simulink model "pmsm_align"  (R2023b)
settings: Solver=FixedStepDiscrete  StartTime=0.0  StopTime=0.05  FixedStep=1e-5  RelTol=1e-3
values from neighbouring files (symbols this model uses):
  V = out.flog.signals.values    [add_ident2.m]    (also in add_w.m; add_w2.m; baseline_model.m; check_kt.m = out.mlog.signals.values)
libraries: spsControlledVoltageSourceLib x3, spsPermanentMagnetSynchronousMachineLib x1, spspowerguiLib x1
settings Model: Creator=28447  LastModifiedBy=28447

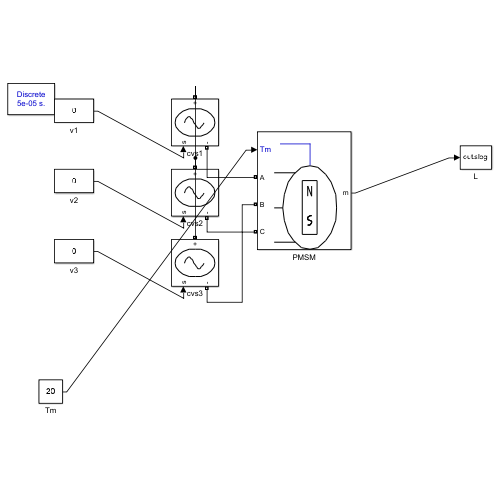
[thumbnail: Simulink's stored preview of the top-level diagram]
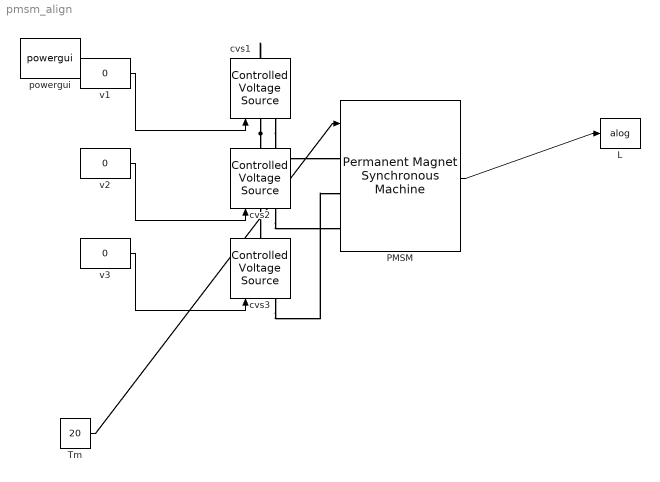
== system pmsm_align ==
  L : ToWorkspace  VariableName=alog  SaveFormat=Structure With Time  SampleTime=-1
  PMSM : spsPermanentMagnetSynchronousMachineLib/Permanent Magnet Synchronous Machine  NbPhases=3  FluxDistribution=Sinusoidal  RotorType=Round  MechanicalLoad=Torque Tm  PresetModel=No  ShowDetailedParameters=on  MeasurementBus=off  Resistance=0.175  Inductance=0.57e-3  dqInductances=[8.5e-3,8.5e-3]  La=0.000395  MachineConstant=Flux linkage established by magnets (V.s)  Flux=0.016833  VoltageCst=12.2127  TorqueCst=0.101  Flat=120  Mechanical=[0.0027 0.0004924 4 0]  PolePairs=4  InitialConditions=[0,0, 0,0]  InitialConditions5ph=[0 0 0 0 0 0]  RefAngle=90 degrees behind phase A axis (modified Park)  IterativeDiscreteModel=Trapezoidal non iterative  TsBlock=-1  TsPowergui=0
  Tm : Constant  Value=20
  cvs1 : spsControlledVoltageSourceLib/Controlled Voltage Source  Initialize=on  Source_Type=AC  Amplitude=0  Phase=0  Frequency=0  Measurements=None
  cvs2 : spsControlledVoltageSourceLib/Controlled Voltage Source  Initialize=on  Source_Type=AC  Amplitude=0  Phase=0  Frequency=0  Measurements=None
  cvs3 : spsControlledVoltageSourceLib/Controlled Voltage Source  Initialize=on  Source_Type=AC  Amplitude=0  Phase=0  Frequency=0  Measurements=None
  powergui : spspowerguiLib/powergui  Priority=1  SimulationMode=Discrete  SampleTime=50e-6  frequency=60  Iterations=50  frequencyindice=60  Pbase=100e6  ErrMax=1e-4  UnitsV=kV  UnitsW=MW  buscounter=0  FunctionMessages=off  echomessages=off  EnableUseOfTLC=off  CurrentSourceSwitches=off  DisableSnubberDevices=off  DisableRonSwitches=off  DisableVfSwitches=off  DisplayEquations=off  AutomaticDiscreteSolvers=off  SolverType=Tustin/Backward Euler (TBE)  Interpol=off  ExternalGateDelay=off  methode=off  Ts=1e-5  x0status=blocks  SPID=on  SwTol=0  HookPort=off  NonlinearTolerance=1e-4  nMaxIteration=100  ContinueOnMaxIteration=off  RestoreLinks=warning  ResistiveCurrentMeasurement=off  Frange=[0:2:500]  Ylog=off  Xlog=on  ShowGrid=off  save=off  variable=ZData  structure=0  ZoomFFT=off  StartTime=0.0  cycles=1  DisplayStyle=1  fundamental=60  FreqAxis=off  MaxFrequency=1000  frequencyindicesteady=1  RmsSteady=1  display=off
  v1 : Constant  Value=0
  v2 : Constant  Value=0
  v3 : Constant  Value=0
  wires:
  v1/1 -> cvs1/1
  v2/1 -> cvs2/1
  v3/1 -> cvs3/1
  Tm/1 -> PMSM/1
  PMSM/1 -> L/1
  connections:
  cvs1/LConn1 -- PMSM/LConn1
  cvs2/LConn1 -- PMSM/LConn2
  cvs3/LConn1 -- PMSM/LConn3
  cvs2/RConn1 -- cvs1/RConn1 -- cvs3/RConn1
